simulink model "tb3_avoid_sl"  (R2025b)
settings: Solver=FixedStepDiscrete  StartTime=0.0  StopTime=inf  FixedStep=0.1  RelTol=1e-3
InitFcn:
  | tb3_sl_stopHook('init');
StopFcn:
  | tb3_sl_stopHook('stop');
model workspace (MAT data in the model file):
  SL_ROS_VariableLengthArrays_MaxSizes.CommonInfo.ArrayTruncateAction = 'EmitWarning'
  SL_ROS_VariableLengthArrays_MaxSizes.MsgTypeMap = containers.Map
  SL_ROS_VariableLengthArrays_MaxSizes.MsgTypeMap.serialization.keys = {'sensor_msgs/LaserScan'}
  SL_ROS_VariableLengthArrays_MaxSizes.MsgTypeMap.serialization.values{1}(1).PropertyName = 'intensities'
  SL_ROS_VariableLengthArrays_MaxSizes.MsgTypeMap.serialization.values{1}(1).DataType = 'single'
  SL_ROS_VariableLengthArrays_MaxSizes.MsgTypeMap.serialization.values{1}(1).MaxLength = 360
  SL_ROS_VariableLengthArrays_MaxSizes.MsgTypeMap.serialization.values{1}(2).PropertyName = 'ranges'
  SL_ROS_VariableLengthArrays_MaxSizes.MsgTypeMap.serialization.values{1}(2).DataType = 'single'
  SL_ROS_VariableLengthArrays_MaxSizes.MsgTypeMap.serialization.values{1}(2).MaxLength = 360
  SL_ROS_VariableLengthArrays_MaxSizes.MsgTypeMap.serialization.uniformity = 0
  SL_ROS_VariableLengthArrays_MaxSizes.MsgTypeMap.serialization.keyType = 'char'
  SL_ROS_VariableLengthArrays_MaxSizes.MsgTypeMap.serialization.valueType = 'any'
values from neighbouring files (symbols this model uses):
  scan = scanSub.LatestMessage    [tb3_avoid.m]    (also in tb3_slam_plan.m = removeInvalidData(scan, "RangeLimits", [0.12 maxRange]))
libraries: ros2lib x3
settings Model: Creator=asus  LastModifiedBy=asus

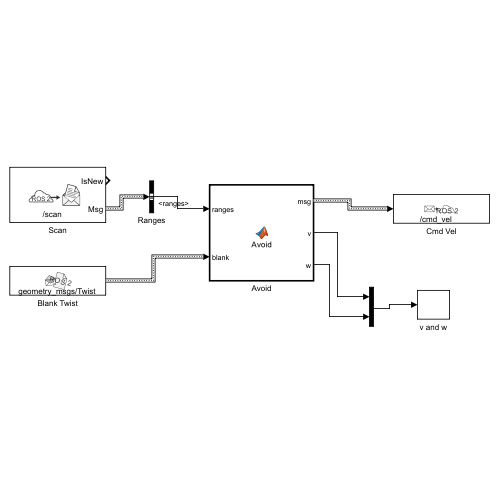
[thumbnail: Simulink's stored preview of the top-level diagram]
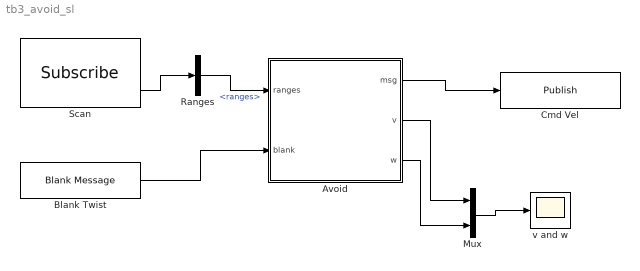
== system tb3_avoid_sl ==
  Avoid : MATLAB Function  TreatAsAtomicUnit=on
  Blank Twist : ros2lib/Blank Message  messageClass=Message  entityType=geometry_msgs/Twist  messageType=geometry_msgs/Twist  SampleTime=inf
  Cmd Vel : ros2lib/Publish  topicSource=Specify your own  topic=/cmd_vel  messageType=geometry_msgs/Twist  QOSHistory=Keep last  QOSDepth=10  QOSReliability=Reliable  QOSDurability=Volatile  QOSDeadline=Inf  QOSLifespan=Inf  QOSLiveliness=Automatic  QOSLeaseDuration=Inf  QOSAvoidROSNamespaceConventions=off
  Mux : Mux  Inputs=2
  Ranges : BusSelector  OutputSignals=ranges
  Scan : ros2lib/Subscribe  topicSource=Specify your own  topic=/scan  messageType=sensor_msgs/LaserScan  sampleTime=0.1  QOSHistory=Keep last  QOSDepth=5  QOSReliability=Best effort  QOSDurability=Volatile  QOSDeadline=Inf  QOSLifespan=Inf  QOSLiveliness=Automatic  QOSLeaseDuration=Inf  QOSAvoidROSNamespaceConventions=off
  v and w : Scope
  wires:
  Scan/2 -> Ranges/1
  Ranges/1 -> Avoid/1(ranges)  "<ranges>"
  Blank Twist/1 -> Avoid/2(blank)
  Avoid/1(msg) -> Cmd Vel/1
  Avoid/2(v) -> Mux/1
  Avoid/3(w) -> Mux/2
  Mux/1 -> v and w/1

== matlab function tb3_avoid_sl/Avoid ==
  data: ranges input; msg output Bus: SL_Bus_geometry_msgs_Twist; blank input Bus: SL_Bus_geometry_msgs_Twist; v output; w output
function [msg, v, w] = Avoid(ranges, blank)
%#codegen
    % /scan 의 ranges 는 single 이고 avoidController 는 double 을 받는다.
    % tb3_avoid.m 에서 double(scan.ranges) 로 넘기는 것과 같다.
    [v, w] = avoidController(double(ranges));

    msg = blank;              % 빈 Twist 를 받아 값만 채운다
    msg.linear.x  = v;
    msg.angular.z = w;
end
